simulink model "eahpSIM"  (R2024b)
settings: Solver=VariableStepAuto  StartTime=0.0  StopTime=5  RelTol=1e-3
values from neighbouring files (symbols this model uses):
  h_filtru = tf(1, [R2 * C2 1])    [init_simulation.m]
  h_integrator = tf(1 / (R1 * C1), [1 0])    [init_simulation.m]
settings Model: Creator=simon  LastModifiedBy=simon

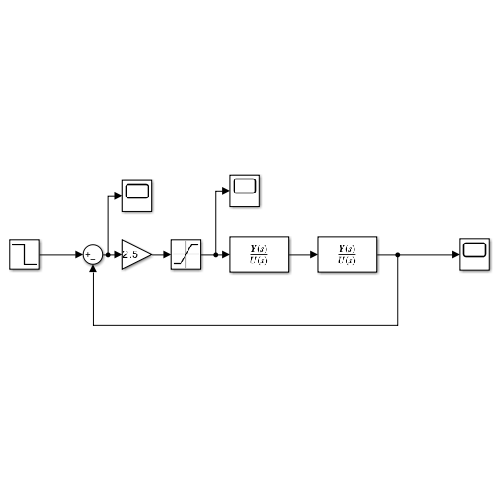
[thumbnail: Simulink's stored preview of the top-level diagram]
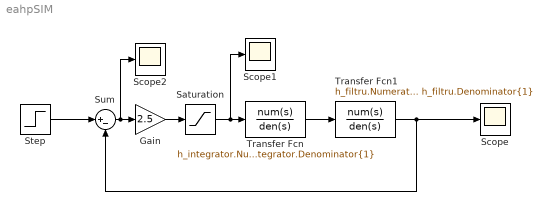
== system eahpSIM ==
  Gain : Gain  Gain=2.5
  Saturation : Saturate  UpperLimit=2.5  LowerLimit=-2.5
  Scope : Scope
  Scope1 : Scope
  Scope2 : Scope
  Step : Step  Time=20  Before=4  After=2  SampleTime=0
  Sum : Sum  Inputs=|+-
  Transfer Fcn : TransferFcn  Numerator=h_integrator.Numerator{1}  Denominator=h_integrator.Denominator{1}
  Transfer Fcn1 : TransferFcn  Numerator=h_filtru.Numerator{1}  Denominator=h_filtru.Denominator{1}
  wires:
  Step/1 -> Sum/1
  Transfer Fcn1/1 -> Sum/2, Scope/1
  Transfer Fcn/1 -> Transfer Fcn1/1
  Sum/1 -> Scope2/1, Gain/1
  Gain/1 -> Saturation/1
  Saturation/1 -> Scope1/1, Transfer Fcn/1
